simulink model "drive_plant_sys"  (R2026b)
settings: Solver=VariableStepAuto
undefined symbols (not defined in the file or in its folder): P
libraries: fl_lib x19, nesl_utility x8, ee_lib x1
settings Model: Creator=aomar  LastModifiedBy=aomar

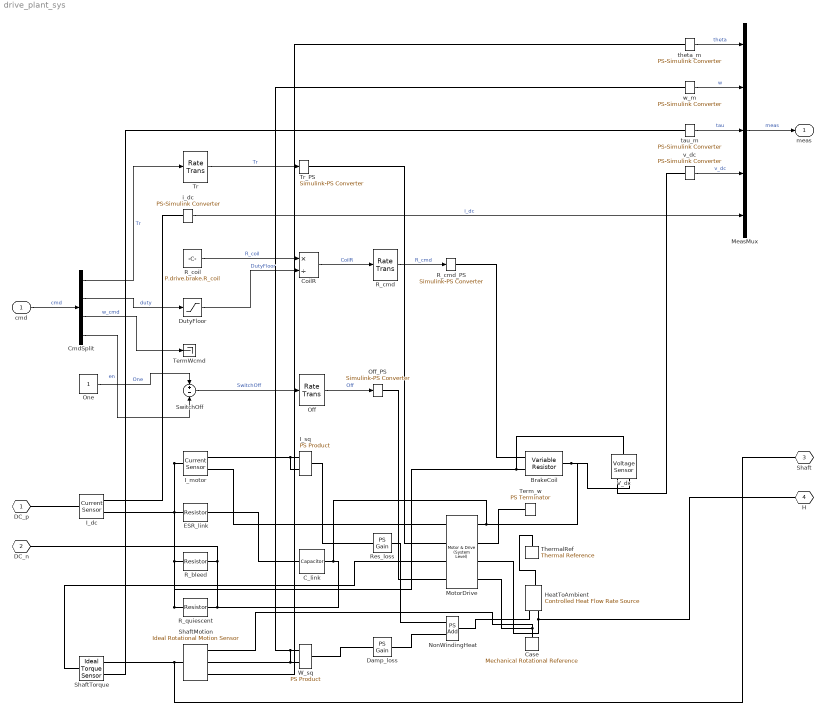
== system drive_plant_sys ==
  cmd : Inport  OutDataTypeStr=double  SampleTime=P.drive.Ts_esc
  BrakeCoil : fl_lib/Electrical/Electrical Elements/Variable Resistor  Rmin=1 Ohm  thermalEnable=false  thermal_mass=1 J/K  i_specify=off  i_priority=None  i=0 A  i_nominal_specify=off  i_nominal_value=1  i_nominal_unit=A  v_specify=off  v_priority=None  v=0 V  v_nominal_specify=off  v_nominal_value=1  v_nominal_unit=V  T_specify=off  T_priority=None  T=300 K  T_nominal_specify=off  T_nominal_value=1  T_nominal_unit=K
  C_link : fl_lib/Electrical/Electrical Elements/Capacitor  c=P.drive.esc.C_link F  r=1e-6 Ohm  g=0 1/Ohm  i_specify=off  i_priority=None  i=0 A  i_nominal_specify=off  i_nominal_value=1  i_nominal_unit=A  v_specify=off  v_priority=None  v=0 V  v_nominal_specify=off  v_nominal_value=1  v_nominal_unit=V  vc_specify=on  vc_priority=High  vc=P.drive.esc.vc0 V  vc_nominal_specify=off  vc_nominal_value=1  vc_nominal_unit=V
  Case : fl_lib/Mechanical/Rotational Elements/Mechanical Rotational Reference
  CmdSplit : Demux
  CoilR : Product  Inputs=*/
  Damp_loss : fl_lib/Physical Signals/Functions/PS Gain  gain=P.drive.motor.lam N*m*s/rad
  DutyFloor : Saturate  UpperLimit=1  LowerLimit=P.drive.brake.duty_min
  ESR_link : fl_lib/Electrical/Electrical Elements/Resistor  R=P.drive.esc.ESR_link Ohm  i_specify=off  i_priority=None  i=0 A  i_nominal_specify=off  i_nominal_value=1  i_nominal_unit=A  v_specify=off  v_priority=None  v=0 V  v_nominal_specify=off  v_nominal_value=1  v_nominal_unit=V
  HeatToAmbient : fl_lib/Thermal/Thermal Sources/Controlled Heat Flow Rate Source
  I_dc : fl_lib/Electrical/Electrical Sensors/Current Sensor
  I_motor : fl_lib/Electrical/Electrical Sensors/Current Sensor
  I_sq : fl_lib/Physical Signals/Functions/PS Product
  MeasMux : Mux  Inputs=5
  MotorDrive : ee_lib/Electromechanical/Motor & Drive (System Level)  torque_speed_param=ee.enum.electromech.envelope.tabulated2D  overtorque_param=ee.enum.electromech.overtorque.no  T_t=[.09, .08, .07, 0] N*m  T_t_intermittent=[.36, .32, .28, 0] N*m  T_t_2D=P.drive.motor.T_pk_2D N*m  T_t_intermittent_2D=[.36, .36, .36; .32, .32, .32; .28, .28, .28; 0, 0, 0] N*m  w_t=P.drive.motor.w_t_rpm rpm  vdc_t=P.drive.motor.vdc_t V  torque_max=0.1 N*m  power_max=30 W  torque_max_intermittent=0.4 N*m  power_max_intermittent=120 W  time_overtorque=30 s  time_recover=60 s  Tc=P.drive.motor.Tc s  EnableSwitch=true  losses_param=ee.enum.electromech.motorAndDrive.lossParameterization.TabulatedLossDataAsAFunctionOfSpeedAndTorque  eff=100  w_eff=3750 rpm  T_eff=0.08 N*m  Piron=0 W  Pbase=0 W  w_eff_vec=P.drive.motor.w_eff_rpm rpm  T_eff_vec=P.drive.motor.T_eff N*m  v_eff_vec=[100, 250, 400] V  losses_mat=P.drive.motor.loss_T1 W  efficiency_mat=[95, 95, 95, 95; 95, 95, 95, 95; 95, 95, 95, 95; 95, 95, 95, 95; 95, 95, 95, 95]  losses_mat_3D=ones(5, 4, 3) W  efficiency_mat_3D=95 * ones(5, 4, 3)  Res=P.drive.motor.Res Ohm  J=P.drive.motor.J kg*m^2  lam=P.drive.motor.lam N*m*s/rad  speed0=0 rpm  faulted_specify=off  faulted_priority=None  faulted=0  faulted_nominal_specify=off  faulted_nominal_value=1  faulted_nominal_unit=1  isSwitchedOff_specify=off  isSwitchedOff_priority=None  isSwitchedOff=0  isSwitchedOff_nominal_specify=off  isSwitchedOff_nominal_value=1  isSwitchedOff_nominal_unit=1  torqueLimitContinuous_specify=off  torqueLimitContinuous_priority=None  torqueLimitContinuous=0 N*m  torqueLimitContinuous_nominal_specify=off  torqueLimitContinuous_nominal_value=1  torqueLimitContinuous_nominal_unit=N*m  TabulateLossesForMultipleTemperatures=false  alpha=3.93e-3 1/K  Tmeas=P.drive.motor.Tmeas1 degC  TmeasVec=[25, 75, 125] degC  Tmeas2=P.drive.motor.Tmeas2 degC  losses_mat_T2=P.drive.motor.loss_T2 W  efficiency_mat_T2=[95, 95, 95, 95; 95, 95, 95, 95; 95, 95, 95, 95; 95, 95, 95, 95; 95, 95, 95, 95]  losses_mat_3D_T2=ones(5, 4, 3) W  efficiency_mat_3D_T2=95 * ones(5, 4, 3)  lossesMatMultipleTemperatures=ones(5, 4, 3) W  efficiencyMatMultipleTemperatures=95 * ones(5, 4, 3)  lossesMat4DMultipleTemperatures=ones(5, 4, 3, 3) W  efficiencyMat4DMultipleTemperatures=95 * ones(5, 4, 3, 3)  thermal_mass=P.drive.thermal.C_w J/K  initial_temperature=P.drive.thermal.T_amb0 K
  NonWindingHeat : fl_lib/Physical Signals/Functions/PS Add
  Off : RateTransition  OutPortSampleTimeOpt=Inherit
  Off_PS : nesl_utility/Simulink-PS Converter  PhysicalDomain=network_engine_domain  SubClassName=ps_input  LeftPortType=input  RightPortType=output  PseudoPeriodic=off  Frequencies=[]  NoiseDistribution=none  NoiseParameters=[]  Unit=1  AffineConversion=off  FilteringAndDerivatives=zero  SimscapeFilterOrder=1  InputFilterTimeConstant=0.001  UdotUserProvided=0
  One : Constant
  R_bleed : fl_lib/Electrical/Electrical Elements/Resistor  R=P.drive.esc.R_bleed Ohm  i_specify=off  i_priority=None  i=0 A  i_nominal_specify=off  i_nominal_value=1  i_nominal_unit=A  v_specify=off  v_priority=None  v=0 V  v_nominal_specify=off  v_nominal_value=1  v_nominal_unit=V
  R_cmd : RateTransition  OutPortSampleTimeOpt=Inherit
  R_cmd_PS : nesl_utility/Simulink-PS Converter  PhysicalDomain=network_engine_domain  SubClassName=ps_input  LeftPortType=input  RightPortType=output  PseudoPeriodic=off  Frequencies=[]  NoiseDistribution=none  NoiseParameters=[]  Unit=Ohm  AffineConversion=off  FilteringAndDerivatives=zero  SimscapeFilterOrder=1  InputFilterTimeConstant=0.001  UdotUserProvided=0
  R_coil : Constant  Value=P.drive.brake.R_coil
  R_quiescent : fl_lib/Electrical/Electrical Elements/Resistor  R=P.drive.esc.R_q Ohm  i_specify=off  i_priority=None  i=0 A  i_nominal_specify=off  i_nominal_value=1  i_nominal_unit=A  v_specify=off  v_priority=None  v=0 V  v_nominal_specify=off  v_nominal_value=1  v_nominal_unit=V
  Res_loss : fl_lib/Physical Signals/Functions/PS Gain  gain=P.drive.motor.Res Ohm
  ShaftMotion : fl_lib/Mechanical/Mechanical Sensors/Ideal Rotational Motion Sensor  reference=foundation.enum.MeasurementReference.difference  acceleration_port=false  velocity_port=true  position_port=true  wrap_angle=false  offset=0 rad
  ShaftTorque : fl_lib/Mechanical/Mechanical Sensors/Ideal Torque Sensor
  SwitchOff : Sum  Inputs=+-
  TermWcmd : Terminator
  Term_w : fl_lib/Physical Signals/Sinks/PS Terminator
  ThermalRef : fl_lib/Thermal/Thermal Elements/Thermal Reference
  Tr : RateTransition  OutPortSampleTimeOpt=Inherit
  Tr_PS : nesl_utility/Simulink-PS Converter  PhysicalDomain=network_engine_domain  SubClassName=ps_input  LeftPortType=input  RightPortType=output  PseudoPeriodic=off  Frequencies=[]  NoiseDistribution=none  NoiseParameters=[]  Unit=N*m  AffineConversion=off  FilteringAndDerivatives=zero  SimscapeFilterOrder=1  InputFilterTimeConstant=0.001  UdotUserProvided=0
  V_dc : fl_lib/Electrical/Electrical Sensors/Voltage Sensor
  W_sq : fl_lib/Physical Signals/Functions/PS Product
  i_dc : nesl_utility/PS-Simulink Converter  PhysicalDomain=network_engine_domain  SubClassName=ps_output  LeftPortType=input  RightPortType=output  PseudoPeriodic=off  Frequencies=[]  VectorFormat=inherit  Unit=A  AffineConversion=off
  tau_m : nesl_utility/PS-Simulink Converter  PhysicalDomain=network_engine_domain  SubClassName=ps_output  LeftPortType=input  RightPortType=output  PseudoPeriodic=off  Frequencies=[]  VectorFormat=inherit  Unit=N*m  AffineConversion=off
  theta_m : nesl_utility/PS-Simulink Converter  PhysicalDomain=network_engine_domain  SubClassName=ps_output  LeftPortType=input  RightPortType=output  PseudoPeriodic=off  Frequencies=[]  VectorFormat=inherit  Unit=rad  AffineConversion=off
  v_dc : nesl_utility/PS-Simulink Converter  PhysicalDomain=network_engine_domain  SubClassName=ps_output  LeftPortType=input  RightPortType=output  PseudoPeriodic=off  Frequencies=[]  VectorFormat=inherit  Unit=V  AffineConversion=off
  w_m : nesl_utility/PS-Simulink Converter  PhysicalDomain=network_engine_domain  SubClassName=ps_output  LeftPortType=input  RightPortType=output  PseudoPeriodic=off  Frequencies=[]  VectorFormat=inherit  Unit=rad/s  AffineConversion=off
  DC_p : PMIOPort  Side=Left  ConnectionType=Connection: foundation.electrical.electrical
  DC_n : PMIOPort  Port=2  Side=Left  ConnectionType=Connection: foundation.electrical.electrical
  Shaft : PMIOPort  Port=3  Side=Right  ConnectionType=Connection: foundation.mechanical.rotational.rotational
  H : PMIOPort  Port=4  Side=Right  ConnectionType=Connection: foundation.thermal.thermal
  meas : Outport  OutDataTypeStr=double
  wires:
  cmd/1 -> CmdSplit/1  "cmd"
  CmdSplit/1 -> Tr/1  "Tr"
  CmdSplit/2 -> DutyFloor/1  "duty"
  CmdSplit/3 -> TermWcmd/1  "w_cmd"
  CmdSplit/4 -> SwitchOff/2  "en"
  One/1 -> SwitchOff/1  "One"
  i_dc/1 -> MeasMux/5  "i_dc"
  SwitchOff/1 -> Off/1  "SwitchOff"
  R_coil/1 -> CoilR/1  "R_coil"
  DutyFloor/1 -> CoilR/2  "DutyFloor"
  Tr/1 -> Tr_PS/1  "Tr"
  CoilR/1 -> R_cmd/1  "CoilR"
  Off/1 -> Off_PS/1  "Off"
  R_cmd/1 -> R_cmd_PS/1  "R_cmd"
  theta_m/1 -> MeasMux/1  "theta"
  w_m/1 -> MeasMux/2  "w"
  tau_m/1 -> MeasMux/3  "tau"
  v_dc/1 -> MeasMux/4  "v_dc"
  MeasMux/1 -> meas/1  "meas"
  connections:
  R_cmd_PS/RConn1 -- BrakeCoil/LConn1
  ESR_link/LConn1 -- I_dc/RConn2 -- I_motor/LConn1 -- R_bleed/LConn1 -- R_quiescent/LConn1 -- BrakeCoil/LConn2 -- V_dc/LConn1
  R_bleed/RConn1 -- DC_n/RConn1 -- R_quiescent/RConn1 -- C_link/RConn1 -- MotorDrive/RConn1 -- BrakeCoil/RConn1 -- V_dc/RConn2
  ESR_link/RConn1 -- C_link/LConn1
  Case/LConn1 -- ShaftMotion/RConn1 -- MotorDrive/RConn4
  DC_p/RConn1 -- I_dc/LConn1
  W_sq/RConn1 -- Damp_loss/LConn1
  Damp_loss/RConn1 -- NonWindingHeat/LConn2
  HeatToAmbient/RConn2 -- MotorDrive/RConn3 -- H/RConn1
  ThermalRef/LConn1 -- HeatToAmbient/LConn1
  NonWindingHeat/RConn1 -- HeatToAmbient/RConn1
  i_dc/LConn1 -- I_dc/RConn1
  I_sq/LConn1 -- I_motor/RConn1 -- I_sq/LConn2
  I_motor/RConn2 -- MotorDrive/LConn1
  I_sq/RConn1 -- Res_loss/LConn1
  Tr_PS/RConn1 -- MotorDrive/LConn2
  ShaftTorque/LConn1 -- MotorDrive/LConn3
  Off_PS/RConn1 -- MotorDrive/LConn4
  MotorDrive/RConn2 -- Term_w/LConn1
  Res_loss/RConn1 -- NonWindingHeat/LConn1
  ShaftMotion/LConn1 -- ShaftTorque/RConn1 -- Shaft/RConn1
  W_sq/LConn1 -- w_m/LConn1 -- W_sq/LConn2 -- ShaftMotion/RConn2
  theta_m/LConn1 -- ShaftMotion/RConn3
  ShaftTorque/RConn2 -- tau_m/LConn1
  v_dc/LConn1 -- V_dc/RConn1
